simulink model "droop_source"  (R2026a)
settings: Solver=ode23t  StopTime=2  MaxStep=5e-5  RelTol=1e-5
model workspace (MAT data in the model file):
  load_L2 = 0.000636619772368
  load_R2 = 0.2
libraries: ee_lib x7, nesl_utility x6, fl_lib x1
settings Model: ModifiedByFormat=GKC3-Simulink contributors  Creator=GKC3-Simulink contributors  LastModifiedBy=GKC3-Simulink contributors

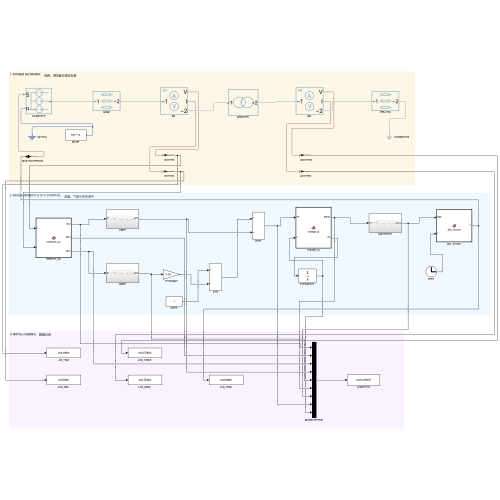
[thumbnail: Simulink's stored preview of the top-level diagram]
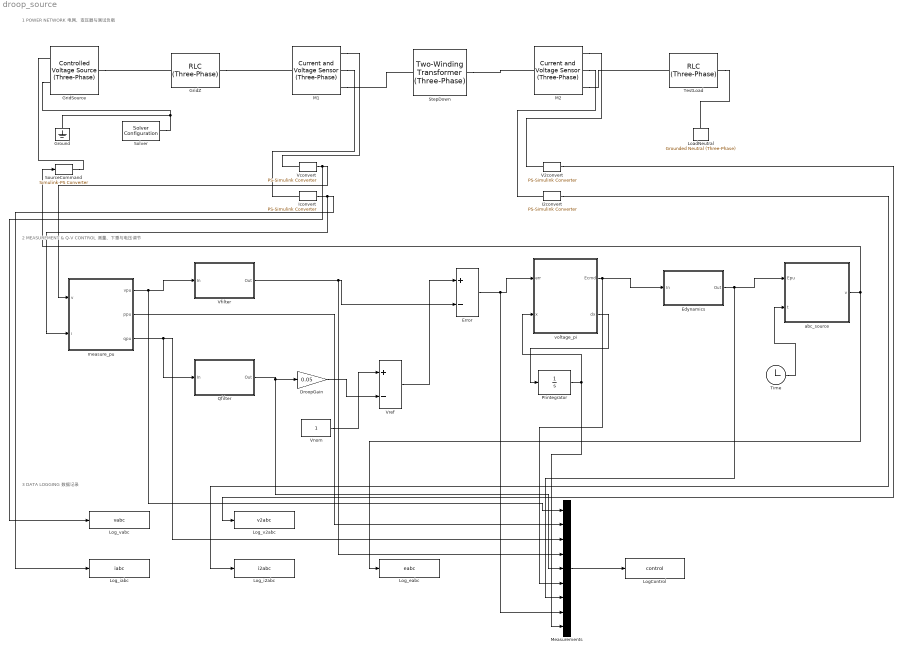
== system droop_source ==
  note: 1 POWER NETWORK 电网、变压器与测试负载
  note: 2 MEASUREMENT & Q-V CONTROL 测量、下垂与电压调节
  note: 3 DATA LOGGING 数据记录
  DroopGain : Gain  Description=Implemented from the task-2 10 kV droop source guide.  Gain=0.05
  Edynamics : Subsystem  Description=Implemented from the task-2 10 kV droop source guide.
  Error : Sum  Description=Implemented from the task-2 10 kV droop source guide.  Inputs=+-
  GridSource : ee_lib/Sources/Controlled Voltage Source (Three-Phase)  Description=Implemented from the task-2 10 kV droop source guide.  input_option=ee.enum.inputType.instantaneous  FRated=50 Hz
  GridZ : ee_lib/Passive/RLC Assemblies/RLC (Three-Phase)  Description=Implemented from the task-2 10 kV droop source guide.  port_option=ee.enum.threePhasePort.composite  component_structure=ee.enum.rlc.structure.SeriesRL  R=0.1961161351 Ohm  L=0.0031212852 H  C=1e-6 F  R_parasitic=0 Ohm  G_parasitic=0 1/Ohm  IL_specify=off  IL_priority=High  IL=[0, 0, 0] A  IL_nominal_specify=off  IL_nominal_value=1  IL_nominal_unit=A  VC_specify=off  VC_priority=High  VC=[0, 0, 0] V  VC_nominal_specify=off  VC_nominal_value=1  VC_nominal_unit=V
  Ground : fl_lib/Electrical/Electrical Elements/Electrical Reference  Description=Implemented from the task-2 10 kV droop source guide.
  I2convert : nesl_utility/PS-Simulink Converter  Description=Implemented from the task-2 10 kV droop source guide.  PhysicalDomain=network_engine_domain  SubClassName=ps_output  LeftPortType=input  RightPortType=output  PseudoPeriodic=off  Frequencies=[]  VectorFormat=inherit  Unit=A  AffineConversion=off
  Iconvert : nesl_utility/PS-Simulink Converter  Description=Implemented from the task-2 10 kV droop source guide.  PhysicalDomain=network_engine_domain  SubClassName=ps_output  LeftPortType=input  RightPortType=output  PseudoPeriodic=off  Frequencies=[]  VectorFormat=inherit  Unit=A  AffineConversion=off
  LoadNeutral : ee_lib/Connectors & References/Grounded Neutral (Three-Phase)  Description=Implemented from the task-2 10 kV droop source guide.  port_option=ee.enum.threePhasePort.composite
  LogControl : ToWorkspace  VariableName=control  SaveFormat=Timeseries  SampleTime=-1
      settings: Description=Implemented from the task-2 10 kV droop source guide.
  Log_eabc : ToWorkspace  VariableName=eabc  SaveFormat=Timeseries  SampleTime=-1
      settings: Description=Implemented from the task-2 10 kV droop source guide.
  Log_i2abc : ToWorkspace  VariableName=i2abc  SaveFormat=Timeseries  SampleTime=-1
      settings: Description=Implemented from the task-2 10 kV droop source guide.
  Log_iabc : ToWorkspace  VariableName=iabc  SaveFormat=Timeseries  SampleTime=-1
      settings: Description=Implemented from the task-2 10 kV droop source guide.
  Log_v2abc : ToWorkspace  VariableName=v2abc  SaveFormat=Timeseries  SampleTime=-1
      settings: Description=Implemented from the task-2 10 kV droop source guide.
  Log_vabc : ToWorkspace  VariableName=vabc  SaveFormat=Timeseries  SampleTime=-1
      settings: Description=Implemented from the task-2 10 kV droop source guide.
  M1 : ee_lib/Sensors & Transducers/Current and Voltage Sensor (Three-Phase)  Description=10 kV bus measurement downstream of grid impedance; current positive toward load.  port_option=ee.enum.threePhasePort.composite  vMeasurementType=ee.enum.vmeasurement.lg  outputUnit=ee.enum.unit.si  SRated=100e6 A*V  VRated=24e3 V  I_specify=off  I_priority=None  I=[0, 0, 0] A  I_nominal_specify=off  I_nominal_value=1  I_nominal_unit=A  V_specify=off  V_priority=None  V=[0, 0, 0] V  V_nominal_specify=off  V_nominal_value=1  V_nominal_unit=V
  M2 : ee_lib/Sensors & Transducers/Current and Voltage Sensor (Three-Phase)  Description=Implemented from the task-2 10 kV droop source guide.  port_option=ee.enum.threePhasePort.composite  vMeasurementType=ee.enum.vmeasurement.lg  outputUnit=ee.enum.unit.si  SRated=100e6 A*V  VRated=24e3 V  I_specify=off  I_priority=None  I=[0, 0, 0] A  I_nominal_specify=off  I_nominal_value=1  I_nominal_unit=A  V_specify=off  V_priority=None  V=[0, 0, 0] V  V_nominal_specify=off  V_nominal_value=1  V_nominal_unit=V
  Measurements : Mux  Description=Implemented from the task-2 10 kV droop source guide.  Inputs=9
  PIintegrator : Integrator  Description=Guide initial condition is 0. Saturation hold test overrides to 0.15 via SimulationInput.
  Qfilter : Subsystem  Description=Implemented from the task-2 10 kV droop source guide.
  Solver : nesl_utility/Solver Configuration  Description=Implemented from the task-2 10 kV droop source guide.  PhysicalDomain=network_engine_domain  SubClassName=solver  LeftPortType=input  RightPortType=generic  Tones=[]  Harmonics=[]  SimulateNoise=off  Profile=off  UseLocalSampling=off  EnableSwitchedLinearOptims=on  FrequencyDomain=off  UseCCode=off  RelTol=0.001  AbsTol=0.001  MinStep=1e-09  ToWorkspace=off  RevertToSquareIcSolve=off  NumHomotopyIterations=100  PhasorMode=off  PhasorModeNumHarmonics=1  ConsistencySolver=NEWTON_XTOL_AFTER_FTOL  CanonicalOrdering=CANONICAL  OptimizeIntermediates=OPTIMIZED  IndexReductionMethod=DerivativeReplacement  DoDC=off  ResidualTolerance=1e-09  ConsistencyTolSource=GLOBAL  ConsistencyAbsTol=0.001  ConsistencyRelTol=0.001  ConsistencyTolFactor=0.001  UseLocalSolver=off  LocalSolverChoice=NE_BACKWARD_EULER_ADVANCER  ResolveIndetEquations=on  FunctionEvalNumThread=1  LocalSolverSampleTime=0.001  DoFixedCost=off  MaxNonlinIter=3  MaxModeIter=2  ComputeImpulses=off  ImpulseIterations=2  LinearAlgebra=auto  LinearAlgebraNumThread=0  EquationFormulation=NE_TIME_EF  DelaysMemoryBudget=1024  AutomaticFiltering=on  FilteringTimeConstant=0.001  PartitionStorageMethod=AS_NEEDED  PartitionMemoryBudget=1024  PartitionMethod=ROBUST  MultibodyUseLocalSolver=off  MultibodyLocalSolverChoice=ODE1  MultibodyLocalSolverSampleTime=0.001
  SourceCommand : nesl_utility/Simulink-PS Converter  Description=Implemented from the task-2 10 kV droop source guide.  PhysicalDomain=network_engine_domain  SubClassName=ps_input  LeftPortType=input  RightPortType=output  PseudoPeriodic=off  Frequencies=[]  NoiseDistribution=none  NoiseParameters=[]  Unit=V  AffineConversion=off  FilteringAndDerivatives=provide  SimscapeFilterOrder=1  InputFilterTimeConstant=0.001  UdotUserProvided=0
  StepDown : ee_lib/Passive/Transformers/Two-Winding Transformer (Three-Phase)  Description=Validation transformer: 10 kV/1000 V, 10 MVA, Yg/Yg, winding R 1e-6 pu each; no leakage/magnetization/saturation.  SRated=10e6 A*V  FRated=50 Hz  Winding1Connection=ee.enum.windingconnection.Yg  VRated1=10000 V  Winding2Connection=ee.enum.windingconnection.Yg  VRated2=1000 V  CoreType=ee.enum.coretype.threelimb  pu_Rw1=1e-6  pu_Rw2=1e-6  leakage_reactance_option=ee.enum.transformer_leakage.exclude  pu_Xl1=0.05  pu_Xl2=0.05  magnetizing_resistance_option=ee.enum.transformer_magnetizingResistance.exclude  pu_Rm=500  magnetizing_reactance_option=ee.enum.transformer_magnetizingReactance.exclude  saturation_option=ee.enum.transformer_saturation.exclude  pu_Xm=500  current_data=[0, .002, 1, 2]  magnetic_flux_data=[0, 1.2, 1.5, 1.51]  pu_X0=0.5  i1_specify=off  i1_priority=None  i1=[0, 0, 0] A  i1_nominal_specify=off  i1_nominal_value=1  i1_nominal_unit=A  i2_specify=off  i2_priority=None  i2=[0, 0, 0] A  i2_nominal_specify=off  i2_nominal_value=1  i2_nominal_unit=A  phi_specify=off  phi_priority=None  phi=[0, 0, 0]  phi_nominal_specify=off  phi_nominal_value=1  phi_nominal_unit=1
  TestLoad : ee_lib/Passive/RLC Assemblies/RLC (Three-Phase)  Description=Validation load. Replace when connecting downstream PWM circuit.  port_option=ee.enum.threePhasePort.composite  component_structure=ee.enum.rlc.structure.SeriesRL  R=load_R2 Ohm  L=load_L2 H  C=1e-6 F  R_parasitic=0 Ohm  G_parasitic=0 1/Ohm  IL_specify=off  IL_priority=High  IL=[0, 0, 0] A  IL_nominal_specify=off  IL_nominal_value=1  IL_nominal_unit=A  VC_specify=off  VC_priority=High  VC=[0, 0, 0] V  VC_nominal_specify=off  VC_nominal_value=1  VC_nominal_unit=V
  Time : Clock
      settings: Description=Implemented from the task-2 10 kV droop source guide.
  V2convert : nesl_utility/PS-Simulink Converter  Description=Implemented from the task-2 10 kV droop source guide.  PhysicalDomain=network_engine_domain  SubClassName=ps_output  LeftPortType=input  RightPortType=output  PseudoPeriodic=off  Frequencies=[]  VectorFormat=inherit  Unit=V  AffineConversion=off
  Vconvert : nesl_utility/PS-Simulink Converter  Description=Implemented from the task-2 10 kV droop source guide.  PhysicalDomain=network_engine_domain  SubClassName=ps_output  LeftPortType=input  RightPortType=output  PseudoPeriodic=off  Frequencies=[]  VectorFormat=inherit  Unit=V  AffineConversion=off
  Vfilter : Subsystem  Description=Implemented from the task-2 10 kV droop source guide.
  Vnom : Constant  Description=Implemented from the task-2 10 kV droop source guide.
  Vref : Sum  Description=Implemented from the task-2 10 kV droop source guide.  Inputs=+-
  abc_source : MATLAB Function  Description=Implemented from the task-2 10 kV droop source guide.  TreatAsAtomicUnit=on
  measure_pu : MATLAB Function  Description=Implemented from the task-2 10 kV droop source guide.  TreatAsAtomicUnit=on
  voltage_pi : MATLAB Function  Description=Implemented from the task-2 10 kV droop source guide.  TreatAsAtomicUnit=on
  wires:
  Measurements/1 -> LogControl/1
  measure_pu/2(ppu) -> Measurements/2
  abc_source/1(v) -> SourceCommand/1, Log_eabc/1
  Time/1 -> abc_source/2(t)
  Edynamics/1(Out) -> abc_source/1(Epu), Measurements/7
  voltage_pi/1(Ecmd) -> Measurements/6, Edynamics/1(In)
  voltage_pi/2(dx) -> PIintegrator/1
  PIintegrator/1 -> Measurements/9, voltage_pi/2(x)
  Error/1 -> Measurements/8, voltage_pi/1(err)
  Vfilter/1(Out) -> Measurements/4, Error/2
  Vref/1 -> Error/1
  Vnom/1 -> Vref/1
  DroopGain/1 -> Vref/2
  Qfilter/1(Out) -> Measurements/5, DroopGain/1
  measure_pu/3(qpu) -> Measurements/3, Qfilter/1(In)
  measure_pu/1(vpu) -> Measurements/1, Vfilter/1(In)
  Iconvert/1 -> Log_iabc/1, measure_pu/2(i)
  Vconvert/1 -> Log_vabc/1, measure_pu/1(v)
  I2convert/1 -> Log_i2abc/1
  V2convert/1 -> Log_v2abc/1
  connections:
  GridSource/LConn2 -- Solver/RConn1 -- Ground/LConn1
  SourceCommand/RConn1 -- GridSource/LConn1
  GridSource/RConn1 -- GridZ/LConn1
  GridZ/RConn1 -- M1/LConn1
  M1/RConn1 -- Vconvert/LConn1
  M1/RConn2 -- Iconvert/LConn1
  M2/RConn2 -- I2convert/LConn1
  M2/RConn1 -- V2convert/LConn1
  M2/RConn3 -- TestLoad/LConn1
  StepDown/RConn1 -- M2/LConn1
  TestLoad/RConn1 -- LoadNeutral/LConn1
  M1/RConn3 -- StepDown/LConn1

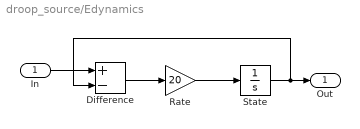
== system droop_source/Edynamics ==
  In : Inport
  Difference : Sum  Inputs=+-
  Rate : Gain  Gain=20
  State : Integrator  InitialCondition=1
  Out : Outport
  wires:
  State/1 -> Difference/2, Out/1
  Rate/1 -> State/1
  Difference/1 -> Rate/1
  In/1 -> Difference/1

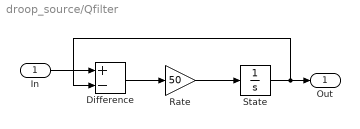
== system droop_source/Qfilter ==
  In : Inport
  Difference : Sum  Inputs=+-
  Rate : Gain  Gain=50
  State : Integrator
  Out : Outport
  wires:
  State/1 -> Difference/2, Out/1
  Rate/1 -> State/1
  Difference/1 -> Rate/1
  In/1 -> Difference/1

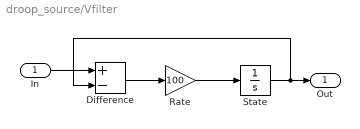
== system droop_source/Vfilter ==
  In : Inport
  Difference : Sum  Inputs=+-
  Rate : Gain  Gain=100
  State : Integrator  InitialCondition=1
  Out : Outport
  wires:
  State/1 -> Difference/2, Out/1
  Rate/1 -> State/1
  Difference/1 -> Rate/1
  In/1 -> Difference/1

== matlab function droop_source/abc_source ==
  data: Epu input; v output; t input
function v = abc_source(Epu,t)
Vll=10000*Epu;
th=2*pi*50*t;
v=sqrt(2/3)*Vll*[sin(th);sin(th-2*pi/3);sin(th+2*pi/3)];
end

== matlab function droop_source/measure_pu ==
  data: v input; vpu output; i input; ppu output; qpu output
function [vpu,ppu,qpu] = measure_pu(v,i)
va=(2/3)*(v(1)-0.5*v(2)-0.5*v(3));
vb=(2/3)*(sqrt(3)/2)*(v(2)-v(3));
ia=(2/3)*(i(1)-0.5*i(2)-0.5*i(3));
ib=(2/3)*(sqrt(3)/2)*(i(2)-i(3));
vpu=sqrt(1.5*(va*va+vb*vb))/10000;
ppu=(v(1)*i(1)+v(2)*i(2)+v(3)*i(3))/1e7;
qpu=1.5*(vb*ia-va*ib)/1e7;
end

== matlab function droop_source/voltage_pi ==
  data: err input; Ecmd output; x input; dx output
function [Ecmd,dx] = voltage_pi(err,x)
raw=0.5*err+x;
u=min(max(raw,-0.15),0.15);
dx=10*err;
if (raw>=0.15 && err>0)||(raw<=-0.15 && err<0)
 dx=0;
end
Ecmd=1+u;
end
